simulink model "wt_twin"  (R2025a)
settings: Solver=FixedStepDiscrete  StartTime=0.0  StopTime=2591400  FixedStep=600  RelTol=1e-3
values from neighbouring files (symbols this model uses):
  T0 = zeros(5, 1)    [run_twin.m]
undefined symbols (not defined in the file or in its folder): a_therm, aero_par, C_therm, k_fault, use_meas
settings Model: Creator=Dhaya  LastModifiedBy=Dhaya

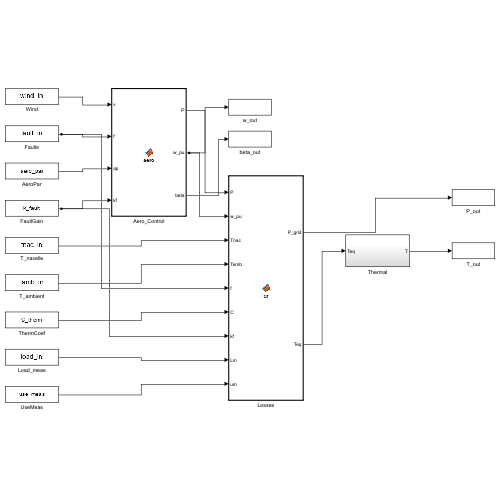
[thumbnail: Simulink's stored preview of the top-level diagram]
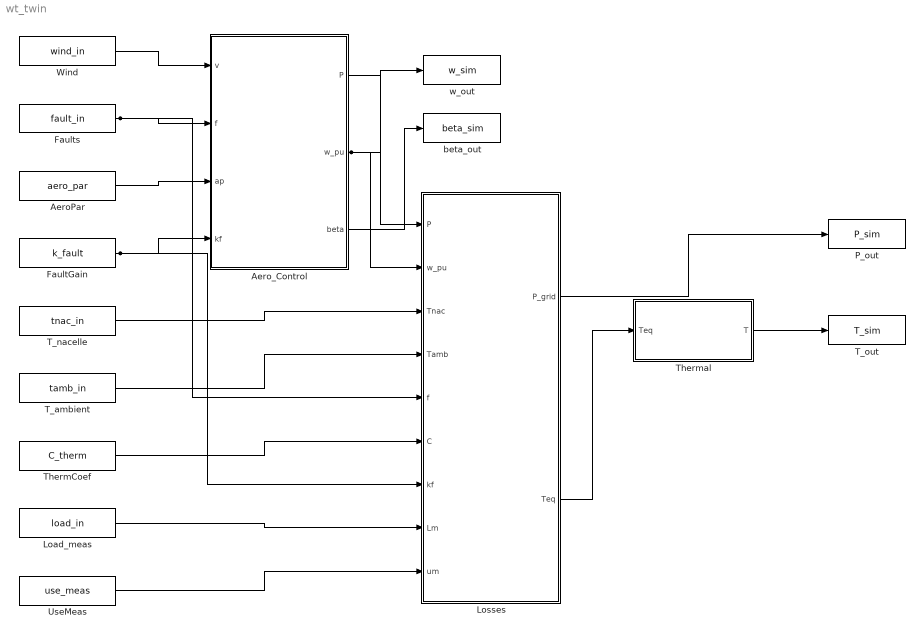
== system wt_twin ==
  AeroPar : Constant  Value=aero_par
  Aero_Control : MATLAB Function  TreatAsAtomicUnit=on
  FaultGain : Constant  Value=k_fault
  Faults : FromWorkspace  VariableName=fault_in  SampleTime=600  Interpolate=off  OutputAfterFinalValue=Holding final value
  Load_meas : FromWorkspace  VariableName=load_in  SampleTime=600  Interpolate=off  OutputAfterFinalValue=Holding final value
  Losses : MATLAB Function  TreatAsAtomicUnit=on
  P_out : ToWorkspace  VariableName=P_sim  SampleTime=600
  T_ambient : FromWorkspace  VariableName=tamb_in  SampleTime=600  Interpolate=off  OutputAfterFinalValue=Holding final value
  T_nacelle : FromWorkspace  VariableName=tnac_in  SampleTime=600  Interpolate=off  OutputAfterFinalValue=Holding final value
  T_out : ToWorkspace  VariableName=T_sim  SampleTime=600
  ThermCoef : Constant  Value=C_therm
  Thermal : Subsystem
  UseMeas : Constant  Value=use_meas
  Wind : FromWorkspace  VariableName=wind_in  SampleTime=600  Interpolate=off  OutputAfterFinalValue=Holding final value
  beta_out : ToWorkspace  VariableName=beta_sim  SampleTime=600
  w_out : ToWorkspace  VariableName=w_sim  SampleTime=600
  wires:
  Wind/1 -> Aero_Control/1(v)
  Faults/1 -> Aero_Control/2(f), Losses/5(f)
  AeroPar/1 -> Aero_Control/3(ap)
  FaultGain/1 -> Aero_Control/4(kf), Losses/7(kf)
  Aero_Control/1(P) -> Losses/1(P)
  Aero_Control/2(w_pu) -> Losses/2(w_pu), w_out/1
  T_nacelle/1 -> Losses/3(Tnac)
  T_ambient/1 -> Losses/4(Tamb)
  ThermCoef/1 -> Losses/6(C)
  Load_meas/1 -> Losses/8(Lm)
  UseMeas/1 -> Losses/9(um)
  Aero_Control/3(beta) -> beta_out/1
  Losses/1(P_grid) -> P_out/1
  Losses/2(Teq) -> Thermal/1(Teq)
  Thermal/1(T) -> T_out/1

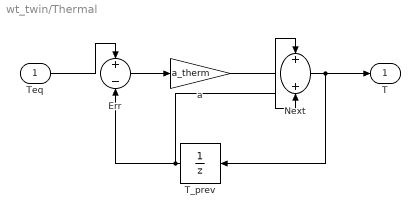
== system wt_twin/Thermal ==
  Teq : Inport
  Err : Sum  Inputs=+-
  Next : Sum
  T_prev : UnitDelay  InitialCondition=T0  SampleTime=600
  a : Gain  Gain=a_therm
  T : Outport
  wires:
  Teq/1 -> Err/1
  T_prev/1 -> Err/2, Next/1
  Err/1 -> a/1
  a/1 -> Next/2
  Next/1 -> T_prev/1, T/1

== matlab function wt_twin/Losses ==
  data: P input; P_grid output; w_pu input; Tnac input; Tamb input; f input; C input; kf input; Lm input; um input; Teq output
function [P_grid, Teq] = losses(P, w_pu, Tnac, Tamb, f, C, kf, Lm, um)
% Component losses -> equilibrium temperatures, with fault injection (see wt_heat.m)
% um = 1: heat from MEASURED power/speed (fault detection, ignores curtailment)
% um = 0: heat from SIMULATED power/speed (pure physics, what-if scenarios)
Pl = P; wl = w_pu;
if um > 0.5, Pl = Lm(1); wl = Lm(2); end
[~, Teq] = wt_heat(Pl, wl, Tnac, Tamb, f, C, kf);
P_grid = P*(1 - kf(2)*f(1));

== matlab function wt_twin/Aero_Control ==
  data: v input; P output; f input; ap input; kf input; w_pu output; beta output
function [P, w_pu, beta] = aero(v, f, ap, kf)
% Rotor aerodynamics + MPPT / pitch control (see wt_aero.m)
% ap = [Kp R wmin Prated Pstandby], hydraulic fault = pitch offset kf(4)*f(3)
[P, w_pu, beta] = wt_aero(v, kf(4)*f(3), ap(1), ap(2), ap(3), ap(4), ap(5));
